simulink model "XorNand"  (R2024b)
settings: Solver=VariableStepAuto  StartTime=0.0  StopTime=inf  RelTol=1e-3
settings Model: Creator=entea  LastModifiedBy=entea

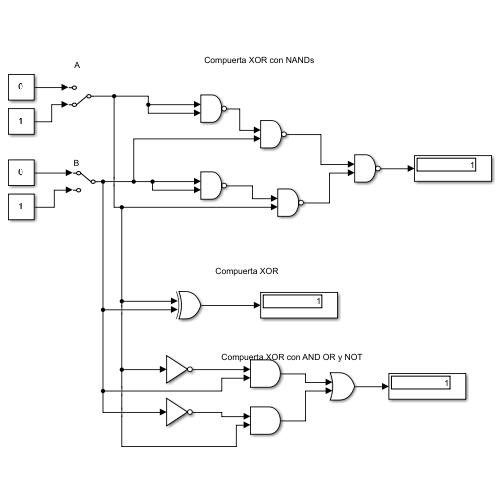
[thumbnail: Simulink's stored preview of the top-level diagram]
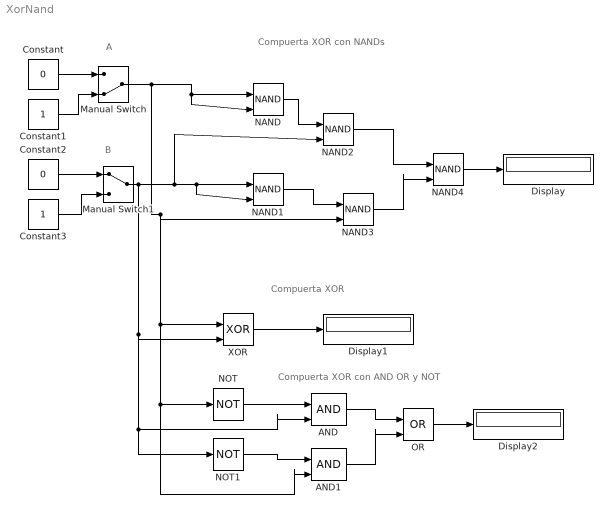
== system XorNand ==
  note: Compuerta XOR con AND OR y NOT
  note: Compuerta XOR
  note: Compuerta XOR con NANDs
  note: B
  note: A
  AND : Logic  IconShape=distinctive  AllPortsSameDT=off  OutDataTypeStr=boolean
  AND1 : Logic  IconShape=distinctive  AllPortsSameDT=off  OutDataTypeStr=boolean
  Constant : Constant  Value=0
  Constant1 : Constant
  Constant2 : Constant  Value=0
  Constant3 : Constant
  Display : Display
  Display1 : Display
  Display2 : Display
  Manual Switch : ManualSwitch  CurrentSetting=0
  Manual Switch1 : ManualSwitch
  NAND{,1..4} (5 alike) : Logic  Operator=NAND  IconShape=distinctive  AllPortsSameDT=off  OutDataTypeStr=boolean
  NOT : Logic  Operator=NOT  IconShape=distinctive  AllPortsSameDT=off  OutDataTypeStr=boolean
  NOT1 : Logic  Operator=NOT  IconShape=distinctive  AllPortsSameDT=off  OutDataTypeStr=boolean
  OR : Logic  Operator=OR  IconShape=distinctive  AllPortsSameDT=off  OutDataTypeStr=boolean
  XOR : Logic  Operator=XOR  IconShape=distinctive  AllPortsSameDT=off  OutDataTypeStr=boolean
  wires:
  Constant/1 -> Manual Switch/1
  Constant1/1 -> Manual Switch/2
  Constant2/1 -> Manual Switch1/1
  Constant3/1 -> Manual Switch1/2
  Manual Switch/1 -> AND1/2, NOT/1, XOR/1, NAND3/2, NAND/2, NAND/1
  Manual Switch1/1 -> AND/2, NOT1/1, XOR/2, NAND2/2, NAND1/2, NAND1/1
  NAND/1 -> NAND2/1
  NAND1/1 -> NAND3/1
  NAND2/1 -> NAND4/1
  NAND3/1 -> NAND4/2
  NAND4/1 -> Display/1
  XOR/1 -> Display1/1
  NOT/1 -> AND/1
  NOT1/1 -> AND1/1
  AND/1 -> OR/1
  AND1/1 -> OR/2
  OR/1 -> Display2/1
